simulink library "roblocks"  (R2019a)
settings: Solver=ode45  StartTime=0.0  StopTime=10  RelTol=1e-3  EnableMultiTasking=on
values from neighbouring files (symbols this model uses):
  q = 1    [quadrotor_plot.m]
undefined symbols (not defined in the file or in its folder): a, angdiff, camera, cinertia, cond, delta2tr, eul2tr, fkine, gravload, inertia, jacob0, jacobe, numcols, P, p560, purepursuit, qd, qdd, qz, rne, robot, rpy2tr, tr2delta, tr2eul, tr2rpy, transl, trnorm, trotz, v_max
(part 2 of 2)

== system roblocks/Vision ==
  note: Cameras
  note: Machine vision
  note: Copyright © 2018 Peter Corke
  note: Machine Vision Toolbox
      | for MATLAB®
  Pose estimation : Subsystem  mask{cam=camera, P=P}
      mask prompts: cam "Camera"; P "Points (3xN)"
      mask help: Pose estimation
      mask Help:
      | Estimate pose of an object based on known 3D points with respect to object
      | coordinate frame, a camera model, and observed object point projections.
      | 
      | <b>Parameters::</b>
      | 
      | Camera (Camera)  The camera object, subclass of Camera class
      | Points (3xN)     The 3D world points in object coordinate frame, one per column
      | 
      | <b>Inputs::</b>
      | 
      | Points (2xN)  The 2D image-plane points, one per column, corresponding
      |               to the columns of Points.
      | 
      | <b>Outputs::</b>
      | 
      | T (4x4) the estimated object pose as a homogeneous transformation
      | 
      | <b>Notes::</b>
      | 
      | - A wrapper for the Toolbox method estpose().
  camera : Subsystem  mask{cam=, points=}
      mask prompts: cam "Camera"; points "Points (3xN)"
      mask help: Camera model
      mask Help:
      | A generalized camera model that projects a set of world points to the image
      | plane.
      | 
      | 
      | <b>Parameters::</b>
      | 
      | Camera (Camera)  The camera object, subclass of Camera class
      | Points (3xN)     The 3D world points, one per column
      | 
      | <b>Inputs::</b>
      | 
      | T (4x4) the camera pose as a homogeneous transformation
      | 
      | 
      | <b>Outputs::</b>
      | 
      | p (2xN) projection of world points, one per column, corresponding to columns
      |         of the parameter Points.
      | 
      | <b>Notes::</b>
      | 
      | - Accepts any camera object derived from the abstract Camera superclass.
  camera1 : Subsystem  mask{cam=0}
      mask prompts: cam "Camera"
      mask help: Camera model for moving object
      mask Help:
      | A generalized camera model that projects a set of world points to the image
      | plane.
      | 
      | 
      | <b>Parameters::</b>
      | 
      | Camera (Camera)  The camera object, subclass of Camera class
      | Points (3xN)     The 3D world points, one per column, with respect to the
      |                  object coordinate frame.
      | 
      | <b>Inputs::</b>
      | 
      | T (4x4)    the camera pose as a homogeneous transformation
      | Tobj (4x4) the pose of the object coordinate frame
      | 
      | <b>Outputs::</b>
      | 
      | p (2xN) projection of world points, one per column, corresponding to columns
      |         of the parameter Points.
      | 
      | <b>Notes::</b>
      | 
      | - This block allows for the object to move, as well as the camera.
      | - Accepts any camera object derived from the abstract Camera superclass.
  camera2 : Subsystem  mask{cam=0, points=0}
      mask prompts: cam "Camera"; points "Points (3xN)"
      mask help: Camera model for moving object
      mask Help:
      | A generalized camera model that projects a set of world points to the image
      | plane.
      | 
      | 
      | <b>Parameters::</b>
      | 
      | Camera (Camera)  The camera object, subclass of Camera class
      | Points (3xN)     The 3D world points, one per column, with respect to the
      |                  object coordinate frame.
      | 
      | <b>Inputs::</b>
      | 
      | T (4x4)    the camera pose as a homogeneous transformation
      | Tobj (4x4) the pose of the object coordinate frame
      | 
      | <b>Outputs::</b>
      | 
      | p (2xN) projection of world points, one per column, corresponding to columns
      |         of the parameter Points.
      | 
      | <b>Notes::</b>
      | 
      | - This block allows for the object to move, as well as the camera.
      | - Accepts any camera object derived from the abstract Camera superclass.
  image Jacobian : Subsystem  mask{cam=, z=}
      mask prompts: cam "Camera"; z "Assumed depth (m)"
      mask help: Image Jacobian
      mask Help:
      | Jacobian matrix relating image plane point velocity to camera spatial
      | velocity expressed in the world frame.
      | 
      | <b>Parameters::</b>
      | 
      | Camera (Camera)  The camera object, subclass of Camera class
      | z (1x1)          Point depth, assumed same for all points
      | z (1xN)          Point depth, unique for each point
      | 
      | <b>Inputs::</b>
      | 
      | Points (2xN)     The 2D image-plane points, one per column
      | 
      | 
      | <b>Outputs::</b>
      | 
      | J (2Nx6) the image Jacobian matrix
      | 
      | <b>Notes::</b>
      | 
      | - For multiple points the Jacobian is the "stack" of the 2x6 point feature
      |   Jacobians.
      | - A wrapper for the Toolbox method visjac_p().

== system roblocks/Arm/RNE ==
  q : Inport
  qd : Inport  Port=2
  qdd : Inport  Port=3
  MATLAB Fcn : MATLABFcn  MATLABFcn=rne(robot, u(1:n)', u(n+1:2*n)', u(2*n+1:3*n)')  OutputDimensions=robot.n
  Mux : Mux  Inputs=3
  Q : Outport
  wires:
  Mux/1 -> MATLAB Fcn/1
  q/1 -> Mux/1
  qd/1 -> Mux/2
  qdd/1 -> Mux/3
  MATLAB Fcn/1 -> Q/1

== system roblocks/Arm/Robot ==
  Q : Inport
  Integrator : Integrator
  Integrator1 : Integrator  InitialCondition=q0
  Mux : Mux  Inputs=3
  S-Function : S-Function  FunctionName=slaccel  Parameters=robot  SFunctionDeploymentMode=off  EnableBusSupport=off
  q : Outport
  qd : Outport  Port=2
  qdd : Outport  Port=3
  wires:
  Integrator1/1 -> Mux/1, q/1
  Q/1 -> Mux/3
  Integrator/1 -> Mux/2, Integrator1/1, qd/1  "qd"
  Mux/1 -> S-Function/1
  S-Function/1 -> Integrator/1, qdd/1  "qdd"

== system roblocks/Arm/cinertia ==
  q : Inport
  cinertia : MATLABFcn  MATLABFcn=cinertia(robot,u')  OutputDimensions=[6 6]  Output1D=off
  Alpha : Outport
  wires:
  cinertia/1 -> Alpha/1
  q/1 -> cinertia/1

== system roblocks/Arm/fkine ==
  q : Inport
  MATLAB Fcn : MATLABFcn  MATLABFcn=double(fkine(robot,u))  OutputDimensions=[4 4]  Output1D=off
  T : Outport
  wires:
  MATLAB Fcn/1 -> T/1
  q/1 -> MATLAB Fcn/1

== system roblocks/Arm/gravload ==
  q : Inport
  gravload : MATLABFcn  MATLABFcn=gravload(robot,u')  OutputDimensions=[1 robot.n]  Output1D=off
  g : Outport
  wires:
  gravload/1 -> g/1
  q/1 -> gravload/1

== system roblocks/Arm/ijacob ==
  J : Inport
  inverse jacobian : MATLABFcn  MATLABFcn=inv(u)  Output1D=off
  Ji : Outport
  wires:
  J/1 -> inverse jacobian/1
  inverse jacobian/1 -> Ji/1

== system roblocks/Arm/ikine ==
  T : Inport
  ikine : MATLABFcn  MATLABFcn=robot.ikine(u, q0, M, opt{:})
  q : Outport
  wires:
  T/1 -> ikine/1
  ikine/1 -> q/1

== system roblocks/Arm/ikine6s ==
  T : Inport
  ikine6s : MATLABFcn  MATLABFcn=robot.ikine6s(u,conf)
  q : Outport
  wires:
  T/1 -> ikine6s/1
  ikine6s/1 -> q/1

== system roblocks/Arm/inertia ==
  q : Inport
  inertia : MATLABFcn  MATLABFcn=inertia(robot,u')  OutputDimensions=[robot.n robot.n]  Output1D=off
  J : Outport
  wires:
  inertia/1 -> J/1
  q/1 -> inertia/1

== system roblocks/Arm/jacob0  ==
  q : Inport
  MATLAB Fcn : MATLABFcn  MATLABFcn=jacob0(robot,u)  OutputDimensions=[6 n]  Output1D=off
  J : Outport
  wires:
  q/1 -> MATLAB Fcn/1
  MATLAB Fcn/1 -> J/1

== system roblocks/Arm/jacobn ==
  q : Inport
  MATLAB Fcn : MATLABFcn  MATLABFcn=jacobe(robot,u)  OutputDimensions=[6 n]  Output1D=off
  J : Outport
  wires:
  q/1 -> MATLAB Fcn/1
  MATLAB Fcn/1 -> J/1

== system roblocks/Arm/plot ==
  q : Inport
  S-Function : S-Function  FunctionName=slplotbot  Parameters=robot,fps,holdplot  SFunctionDeploymentMode=off  EnableBusSupport=off
  fps : ZeroOrderHold  SampleTime=1/fps
  wires:
  fps/1 -> S-Function/1
  q/1 -> fps/1

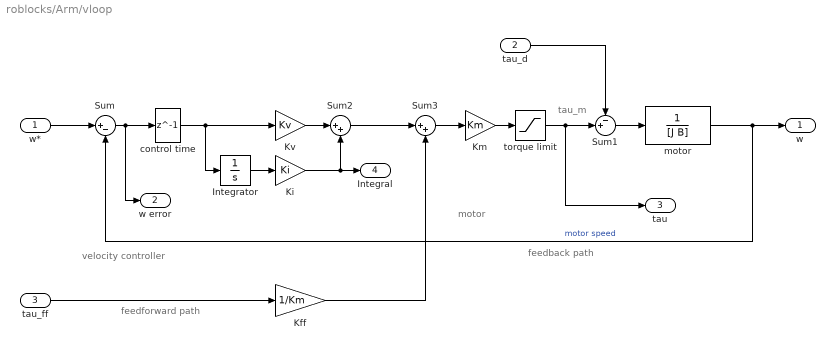
== system roblocks/Arm/vloop ==
  note: feedback path
  note: motor
  note: tau_m
  note: feedforward path
  note: velocity controller
  w* : Inport
  tau_d : Inport  Port=2
  tau_ff : Inport  Port=3
  Integrator : Integrator
  Kff : Gain  Gain=1/Km
  Ki : Gain  Gain=Ki
  Km : Gain  Gain=Km
  Kv : Gain  Gain=Kv
  Sum : Sum  Inputs=|+-
  Sum1 : Sum  Inputs=-+|
  Sum2 : Sum  Inputs=|++
  Sum3 : Sum  Inputs=|++
  control time : Delay  DelayLength=1  SampleTime=T
  motor : TransferFcn  Denominator=[J B]  ContinuousStateAttributes='qd'
  torque limit : Saturate  UpperLimit=tau_max  LowerLimit=-tau_max
  w : Outport
  w error : Outport  Port=2
  tau : Outport  Port=3
  Integral : Outport  Port=4
  wires:
  Sum1/1 -> motor/1
  Sum/1 -> control time/1, w error/1
  motor/1 -> w/1, Sum/2  "motor speed"
  tau_d/1 -> Sum1/1
  torque limit/1 -> Sum1/2, tau/1
  control time/1 -> Kv/1, Integrator/1
  w*/1 -> Sum/1
  Km/1 -> torque limit/1
  Kv/1 -> Sum2/1
  Integrator/1 -> Ki/1
  Ki/1 -> Integral/1, Sum2/2
  Sum2/1 -> Sum3/1
  Sum3/1 -> Km/1
  Kff/1 -> Sum3/2
  tau_ff/1 -> Kff/1

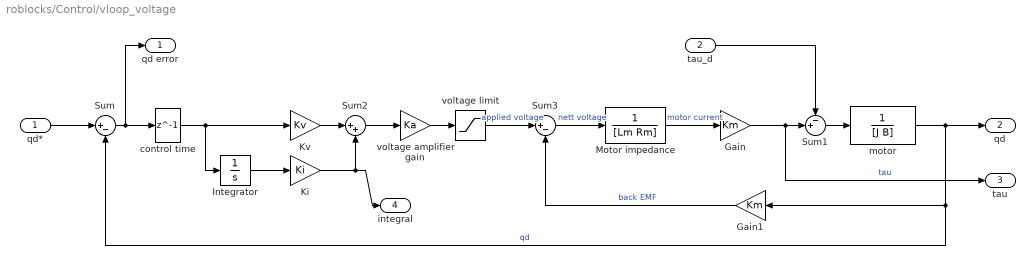
== system roblocks/Control/vloop_voltage ==
  qd* : Inport
  tau_d : Inport  Port=2
  Gain : Gain  Gain=Km
  Gain1 : Gain  Gain=Km
  Integrator : Integrator
  Ki : Gain  Gain=Ki
  Kv : Gain  Gain=Kv
  Motor impedance : TransferFcn  Denominator=[Lm Rm]
  Sum : Sum  Inputs=|+-
  Sum1 : Sum  Inputs=-+|
  Sum2 : Sum  Inputs=|++
  Sum3 : Sum  Inputs=|+-
  control time : Delay  DelayLength=1  SampleTime=T
  motor : TransferFcn  Denominator=[J B]  ContinuousStateAttributes='qd'
  voltage amplifier gain : Gain  Gain=Ka
  voltage limit : Saturate  UpperLimit=v_max  LowerLimit=-v_max
  qd error : Outport
  qd : Outport  Port=2
  tau : Outport  Port=3
  integral : Outport  Port=4
  wires:
  Gain1/1 -> Sum3/2  "back EMF"
  Gain/1 -> tau/1, Sum1/2  "tau"
  Motor impedance/1 -> Gain/1  "motor current"
  Sum3/1 -> Motor impedance/1  "nett voltage"
  voltage limit/1 -> Sum3/1  "applied voltage"
  voltage amplifier gain/1 -> voltage limit/1
  Ki/1 -> integral/1, Sum2/2
  Integrator/1 -> Ki/1
  Kv/1 -> Sum2/1
  Sum2/1 -> voltage amplifier gain/1
  qd*/1 -> Sum/1
  control time/1 -> Integrator/1, Kv/1
  tau_d/1 -> Sum1/1
  motor/1 -> Gain1/1, Sum/2, qd/1  "qd"
  Sum/1 -> qd error/1, control time/1
  Sum1/1 -> motor/1

== system roblocks/Toolbox/Circle ==
  Clock : Clock
  Mux : Mux  Inputs=2
  Product1 : Product  RndMeth=Zero
  Trigonometric Function1 : Trigonometry  Operator=cos
  Trigonometric Function3 : Trigonometry
  freq : Gain  Gain=freq*2*pi
  radius : Constant  Value=radius
  xy : Outport
  wires:
  Trigonometric Function3/1 -> Mux/2
  Trigonometric Function1/1 -> Mux/1
  Mux/1 -> Product1/1
  radius/1 -> Product1/2
  Clock/1 -> freq/1
  Product1/1 -> xy/1
  freq/1 -> Trigonometric Function1/1, Trigonometric Function3/1

== system roblocks/Toolbox/Inverse ==
  T : Inport
  MATLAB Fcn : MATLABFcn  MATLABFcn=inv(u)  OutputDimensions=[4,4]  Output1D=off
  invT : Outport
  wires:
  MATLAB Fcn/1 -> invT/1
  T/1 -> MATLAB Fcn/1

== system roblocks/Toolbox/Post multiply ==
  T1 : Inport
  Constant : Constant  Value=T2
  Product : Product  Multiplication=Matrix(*)  RndMeth=Zero
  T : Outport
  wires:
  T1/1 -> Product/1
  Constant/1 -> Product/2
  Product/1 -> T/1

== system roblocks/Toolbox/Pre multiply ==
  T2 : Inport
  Constant : Constant  Value=T  VectorParams1D=off
  Product : Product  Multiplication=Matrix(*)  RndMeth=Zero
  T : Outport
  wires:
  T2/1 -> Product/2
  Product/1 -> T/1
  Constant/1 -> Product/1

== system roblocks/Toolbox/SE2 to SE3 ==
  SE2 : Inport
  SE2->SE3 : MATLABFcn  MATLABFcn=transl(u(1), u(2), 0)*trotz(u(3))  Output1D=off
  T : Outport
  wires:
  SE2->SE3/1 -> T/1
  SE2/1 -> SE2->SE3/1

== system roblocks/Toolbox/T2eul ==
  T : Inport
  Demux : Demux  Outputs=3
  MATLAB Fcn : MATLABFcn  MATLABFcn=tr2eul(u, args{:})  OutputDimensions=3
  a : Outport
  b : Outport  Port=2
  c : Outport  Port=3
  wires:
  T/1 -> MATLAB Fcn/1
  MATLAB Fcn/1 -> Demux/1
  Demux/1 -> a/1
  Demux/2 -> b/1
  Demux/3 -> c/1

== system roblocks/Toolbox/T2rpy ==
  T : Inport
  Demux : Demux  Outputs=3
  MATLAB Fcn : MATLABFcn  MATLABFcn=tr2rpy(u, args{:})  OutputDimensions=3
  roll : Outport
  pitch : Outport  Port=2
  yaw : Outport  Port=3
  wires:
  T/1 -> MATLAB Fcn/1
  MATLAB Fcn/1 -> Demux/1
  Demux/1 -> roll/1
  Demux/2 -> pitch/1
  Demux/3 -> yaw/1

== system roblocks/Toolbox/T2xyz ==
  T : Inport
  Demux : Demux  Outputs=3
  MATLAB Fcn : MATLABFcn  MATLABFcn=transl(u)  OutputDimensions=3
  x : Outport
  y : Outport  Port=2
  z : Outport  Port=3
  wires:
  Demux/3 -> z/1
  Demux/2 -> y/1
  Demux/1 -> x/1
  MATLAB Fcn/1 -> Demux/1
  T/1 -> MATLAB Fcn/1

== system roblocks/Toolbox/angdiff ==
  + : Inport
  - : Inport  Port=2
  MATLAB Fcn : MATLABFcn  MATLABFcn=angdiff(u(1), u(2))
  Mux : Mux  Inputs=2
  d : Outport
  wires:
  -/1 -> Mux/2
  MATLAB Fcn/1 -> d/1
  Mux/1 -> MATLAB Fcn/1
  +/1 -> Mux/1

== system roblocks/Toolbox/angdiff1 ==
  + : Inport
  MATLAB Fcn : MATLABFcn  MATLABFcn=angdiff(u)
  d : Outport
  wires:
  MATLAB Fcn/1 -> d/1
  +/1 -> MATLAB Fcn/1

== system roblocks/Toolbox/eul2T ==
  a : Inport
  b : Inport  Port=2
  c : Inport  Port=3
  MATLAB Fcn : MATLABFcn  MATLABFcn=eul2tr(u', args{:})  OutputDimensions=[4 4]  Output1D=off
  Mux : Mux  Inputs=3
  T : Outport
  wires:
  b/1 -> Mux/2
  a/1 -> Mux/1
  Mux/1 -> MATLAB Fcn/1
  MATLAB Fcn/1 -> T/1
  c/1 -> Mux/3

== system roblocks/Toolbox/invJac ==
  J : Inport
  e : Inport  Port=2
  MATLAB Fcn2 : MATLABFcn  MATLABFcn=cond(u)  Output1D=off
  Product1 : Product  Multiplication=Matrix(*)  SaturateOnIntegerOverflow=on  RndMeth=Zero  InputSameDT=on  OutDataTypeStr=Inherit: Same as first input
  inv : MATLABFcn  MATLABFcn=pinv(u)  Output1D=off
  vdot : Outport
  cond : Outport  Port=2
  wires:
  Product1/1 -> vdot/1
  MATLAB Fcn2/1 -> cond/1
  e/1 -> Product1/2
  inv/1 -> Product1/1
  J/1 -> inv/1, MATLAB Fcn2/1

== system roblocks/Toolbox/jtraj ==
  Clock : Clock
  MATLAB Fcn : MATLABFcn  MATLABFcn=interp1(t,q,min(u,tmax))  OutputDimensions=n  SampleTime=ts
  MATLAB Fcn1 : MATLABFcn  MATLABFcn=interp1(t,qd,min(u,tmax))  OutputDimensions=n  SampleTime=ts
  MATLAB Fcn2 : MATLABFcn  MATLABFcn=interp1(t,qdd,min(u,tmax))  OutputDimensions=n  SampleTime=ts
  q : Outport
  qd : Outport  Port=2
  qdd : Outport  Port=3
  wires:
  MATLAB Fcn2/1 -> qdd/1
  Clock/1 -> MATLAB Fcn2/1, MATLAB Fcn1/1, MATLAB Fcn/1
  MATLAB Fcn1/1 -> qd/1
  MATLAB Fcn/1 -> q/1

== system roblocks/Toolbox/lspb ==
  Clock : Clock
  MATLAB Fcn : MATLABFcn  MATLABFcn=interp1(t,q,u)  OutputDimensions=n
  MATLAB Fcn1 : MATLABFcn  MATLABFcn=interp1(t,qd,u)  OutputDimensions=n
  MATLAB Fcn2 : MATLABFcn  MATLABFcn=interp1(t,qdd,u)  OutputDimensions=n
  q : Outport
  qd : Outport  Port=2
  qdd : Outport  Port=3
  wires:
  MATLAB Fcn/1 -> q/1
  MATLAB Fcn1/1 -> qd/1
  Clock/1 -> MATLAB Fcn/1, MATLAB Fcn1/1, MATLAB Fcn2/1
  MATLAB Fcn2/1 -> qdd/1

== system roblocks/Toolbox/mstraj ==
  Clock : Clock
  Interpreted MATLAB Function : MATLABFcn  MATLABFcn=interp1( linspace(0, total_time, size(robot_traj,1)), robot_traj, u)
  xy : Outport
  wires:
  Clock/1 -> Interpreted MATLAB Function/1
  Interpreted MATLAB Function/1 -> xy/1

== system roblocks/Toolbox/norm ==
  v : Inport
  norm : MATLABFcn  MATLABFcn=norm(u)
  n : Outport
  wires:
  norm/1 -> n/1
  v/1 -> norm/1

== system roblocks/Toolbox/pinvJac ==
  J : Inport
  e : Inport  Port=2
  MATLAB Fcn2 : MATLABFcn  MATLABFcn=cond(u)  Output1D=off
  Product1 : Product  Multiplication=Matrix(*)  SaturateOnIntegerOverflow=on  RndMeth=Zero  InputSameDT=on  OutDataTypeStr=Inherit: Same as first input
  pinv : MATLABFcn  MATLABFcn=pinv(u)  Output1D=off
  vdot : Outport
  cond : Outport  Port=2
  wires:
  Product1/1 -> vdot/1
  MATLAB Fcn2/1 -> cond/1
  e/1 -> Product1/2
  pinv/1 -> Product1/1
  J/1 -> pinv/1, MATLAB Fcn2/1

== system roblocks/Toolbox/pose integral ==
  v : Inport
  MATLAB Fcn3 : MATLABFcn  MATLABFcn=delta2tr(u*dt)  Output1D=off
  Product : Product  Multiplication=Matrix(*)  RndMeth=Zero
  Unit Delay : UnitDelay  InitialCondition=T0  SampleTime=dt  HasFrameUpgradeWarning=on
  trnorm : MATLABFcn  MATLABFcn=trnorm(u)  Output1D=off
  T : Outport
  wires:
  v/1 -> MATLAB Fcn3/1
  trnorm/1 -> Unit Delay/1
  MATLAB Fcn3/1 -> Product/1
  Unit Delay/1 -> T/1, Product/2
  Product/1 -> trnorm/1

== system roblocks/Toolbox/pure pursuit ==
  CP : Inport
  Interpreted MATLAB Function : MATLABFcn  MATLABFcn=purepursuit(u, R, robot_traj)
  PP : Outport
  wires:
  CP/1 -> Interpreted MATLAB Function/1
  Interpreted MATLAB Function/1 -> PP/1

== system roblocks/Toolbox/rpy2T ==
  roll : Inport
  pitch : Inport  Port=2
  yaw : Inport  Port=3
  MATLAB Fcn : MATLABFcn  MATLABFcn=rpy2tr(u', args{:})  OutputDimensions=[4 4]  Output1D=off
  Mux : Mux  Inputs=3
  T : Outport
  wires:
  pitch/1 -> Mux/2
  roll/1 -> Mux/1
  Mux/1 -> MATLAB Fcn/1
  MATLAB Fcn/1 -> T/1
  yaw/1 -> Mux/3

== system roblocks/Toolbox/tr2delta ==
  T1 : Inport
  T2 : Inport  Port=2
  MATLAB Fcn : MATLABFcn  MATLABFcn=tr2delta(reshape(u(1:16),4,4), reshape(u(17:32),4,4))  OutputDimensions=6
  Mux : Mux  Inputs=2
  Reshape : Reshape
  Reshape1 : Reshape
  delta : Outport
  wires:
  Reshape1/1 -> Mux/2
  Reshape/1 -> Mux/1
  Mux/1 -> MATLAB Fcn/1
  T2/1 -> Reshape1/1
  T1/1 -> Reshape/1
  MATLAB Fcn/1 -> delta/1

== system roblocks/Toolbox/tr2diff ==
  T1 : Inport
  T2 : Inport  Port=2
  MATLAB Fcn : MATLABFcn  MATLABFcn=tr2delta(reshape(u(1:16),4,4), reshape(u(17:32),4,4))  OutputDimensions=6
  Mux : Mux  Inputs=2
  Reshape : Reshape
  Reshape1 : Reshape
  dx : Outport
  wires:
  Reshape1/1 -> Mux/2
  Reshape/1 -> Mux/1
  Mux/1 -> MATLAB Fcn/1
  T2/1 -> Reshape1/1
  T1/1 -> Reshape/1
  MATLAB Fcn/1 -> dx/1

== system roblocks/Toolbox/trprint ==
  T : Inport
  S-Function : S-Function  FunctionName=sltrprint  Parameters=options  SFunctionDeploymentMode=off  EnableBusSupport=off
  wires:
  T/1 -> S-Function/1

== system roblocks/Toolbox/xyt to SE3 ==
  x : Inport
  y : Inport  Port=2
  theta : Inport  Port=3
  Mux : Mux  Inputs=3
  SE2->SE3 : MATLABFcn  MATLABFcn=transl(u(1), u(2), 0)*trotz(u(3))  Output1D=off
  T : Outport
  wires:
  Mux/1 -> SE2->SE3/1
  y/1 -> Mux/2
  x/1 -> Mux/1
  theta/1 -> Mux/3
  SE2->SE3/1 -> T/1

== system roblocks/Toolbox/xyz2T ==
  x : Inport
  y : Inport  Port=2
  z : Inport  Port=3
  MATLAB Fcn : MATLABFcn  MATLABFcn=transl(u)  OutputDimensions=[4 4]  Output1D=off
  Mux : Mux  Inputs=3
  T : Outport
  wires:
  z/1 -> Mux/3
  MATLAB Fcn/1 -> T/1
  Mux/1 -> MATLAB Fcn/1
  x/1 -> Mux/1
  y/1 -> Mux/2

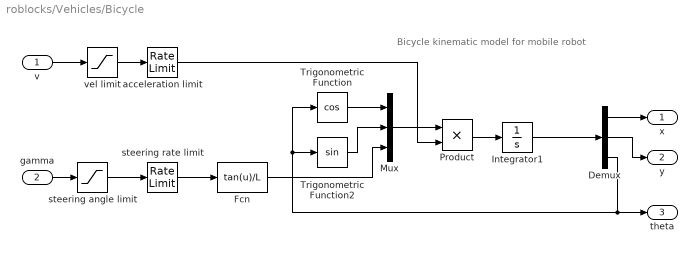
== system roblocks/Vehicles/Bicycle ==
  note: Bicycle kinematic model for mobile robot
  v : Inport
  gamma : Inport  Port=2
  Demux : Demux  Outputs=3
  Fcn : Fcn  Expr=tan(u)/L
  Integrator1 : Integrator  InitialCondition=x0
  Mux : Mux  Inputs=3
  Product : Product  RndMeth=Zero
  Trigonometric Function : Trigonometry  Operator=cos
  Trigonometric Function2 : Trigonometry
  acceleration limit : RateLimiter  RisingSlewLimit=accel  FallingSlewLimit=-accel  SampleTimeMode=inherited
  steering angle limit : Saturate  UpperLimit=alim  LowerLimit=-alim
  steering rate limit : RateLimiter  RisingSlewLimit=steer_rate  FallingSlewLimit=-steer_rate  SampleTimeMode=inherited
  vel limit : Saturate  UpperLimit=vlim  LowerLimit=-vlim
  x : Outport
  y : Outport  Port=2
  theta : Outport  Port=3
  wires:
  steering angle limit/1 -> steering rate limit/1
  Trigonometric Function2/1 -> Mux/2
  vel limit/1 -> acceleration limit/1
  Mux/1 -> Product/1
  v/1 -> vel limit/1
  gamma/1 -> steering angle limit/1
  Demux/2 -> y/1
  Demux/1 -> x/1
  Demux/3 -> theta/1, Trigonometric Function2/1, Trigonometric Function/1
  acceleration limit/1 -> Product/2
  Trigonometric Function/1 -> Mux/1
  Fcn/1 -> Mux/3
  Integrator1/1 -> Demux/1
  Product/1 -> Integrator1/1
  steering rate limit/1 -> Fcn/1

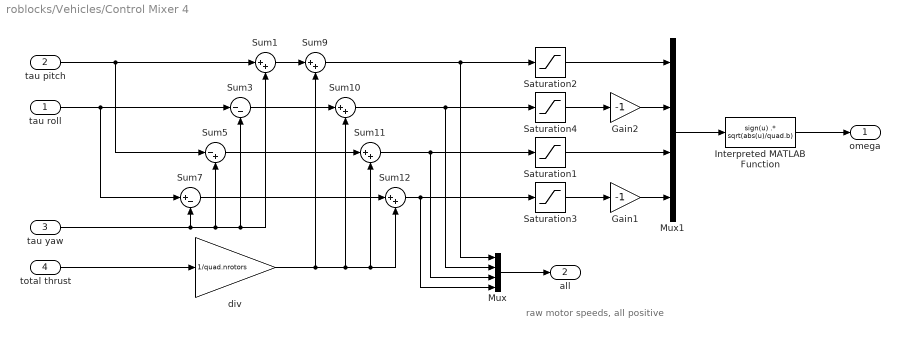
== system roblocks/Vehicles/Control Mixer 4 ==
  note: raw motor speeds, all positive
  tau roll : Inport
  tau pitch : Inport  Port=2
  tau yaw : Inport  Port=3
  total thrust : Inport  Port=4
  Gain1 : Gain  Gain=-1
  Gain2 : Gain  Gain=-1
  Interpreted MATLAB Function : MATLABFcn  MATLABFcn=sign(u) .* sqrt(abs(u)/quad.b)
  Mux : Mux
  Mux1 : Mux
  Saturation{1..4} (4 alike) : Saturate  UpperLimit=maxrot  LowerLimit=minrot
  Sum{1,9..12} (5 alike) : Sum  Inputs=|++  SaturateOnIntegerOverflow=on  InputSameDT=on  OutDataTypeStr=Inherit: Same as first input
  Sum3 : Sum  Inputs=|--  SaturateOnIntegerOverflow=on  InputSameDT=on  OutDataTypeStr=Inherit: Same as first input
  Sum5 : Sum  Inputs=|-+  SaturateOnIntegerOverflow=on  InputSameDT=on  OutDataTypeStr=Inherit: Same as first input
  Sum7 : Sum  Inputs=|+-  SaturateOnIntegerOverflow=on  InputSameDT=on  OutDataTypeStr=Inherit: Same as first input
  div : Gain  Gain=1/quad.nrotors
  omega : Outport
  all : Outport  Port=2
  wires:
  Gain1/1 -> Mux1/4
  Mux/1 -> all/1
  tau roll/1 -> Sum7/1, Sum3/1
  total thrust/1 -> div/1
  Sum12/1 -> Saturation3/1, Mux/4
  Sum11/1 -> Saturation1/1, Mux/3
  Sum10/1 -> Saturation4/1, Mux/2
  Sum9/1 -> Mux/1, Saturation2/1
  Sum7/1 -> Sum12/1
  Sum5/1 -> Sum11/1
  Sum3/1 -> Sum10/1
  Sum1/1 -> Sum9/1
  tau pitch/1 -> Sum5/1, Sum1/1
  Saturation3/1 -> Gain1/1
  Saturation1/1 -> Mux1/3
  Saturation4/1 -> Gain2/1
  Saturation2/1 -> Mux1/1
  tau yaw/1 -> Sum1/2, Sum3/2, Sum5/2, Sum7/2
  Gain2/1 -> Mux1/2
  Mux1/1 -> Interpreted MATLAB Function/1
  Interpreted MATLAB Function/1 -> omega/1
  div/1 -> Sum9/2, Sum10/2, Sum12/2, Sum11/2

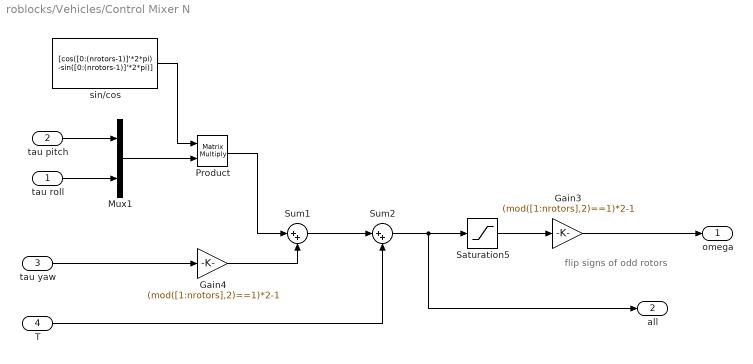
== system roblocks/Vehicles/Control Mixer N ==
  note: flip signs of odd rotors
  tau roll : Inport
  tau pitch : Inport  Port=2
  tau yaw : Inport  Port=3
  T : Inport  Port=4
  Gain3 : Gain  Gain=(mod([1:nrotors],2)==1)*2-1
  Gain4 : Gain  Gain=(mod([1:nrotors],2)==1)*2-1
  Mux1 : Mux  Inputs=2
  Product : Product  Multiplication=Matrix(*)
  Saturation5 : Saturate  UpperLimit=wmax  LowerLimit=wmin
  Sum1 : Sum  Inputs=|++  SaturateOnIntegerOverflow=on  InputSameDT=on  OutDataTypeStr=Inherit: Same as first input
  Sum2 : Sum  Inputs=|++  SaturateOnIntegerOverflow=on  InputSameDT=on  OutDataTypeStr=Inherit: Same as first input
  sin/cos : Constant  Value="[cos([0:(nrotors-1)]'*2*pi)  -sin([0:(nrotors-1)]'*2*pi)]"  VectorParams1D=off  SampleTime=0
  omega : Outport
  all : Outport  Port=2
  wires:
  tau roll/1 -> Mux1/2
  Sum2/1 -> all/1, Saturation5/1
  Saturation5/1 -> Gain3/1
  T/1 -> Sum2/2
  Sum1/1 -> Sum2/1
  tau yaw/1 -> Gain4/1
  Gain4/1 -> Sum1/2
  Gain3/1 -> omega/1
  tau pitch/1 -> Mux1/1
  Mux1/1 -> Product/2
  sin/cos/1 -> Product/1
  Product/1 -> Sum1/1

== system roblocks/Vehicles/N-rotor ==
  omega : Inport
  Bus Creator : BusCreator  Inputs='X','Y','Z','yaw','pitch','roll','dx','dy','dz','dyaw','dpitch','droll'
  Demux : Demux  Outputs=12
  Dynamics : S-Function  FunctionName=nrotor_dynamics  Parameters=quad, x0, ground  SFunctionDeploymentMode=off  EnableBusSupport=off
  X : Outport
  wires:
  Demux/12 -> Bus Creator/12  "droll"
  Demux/11 -> Bus Creator/11  "dpitch"
  Demux/10 -> Bus Creator/10  "dyaw"
  Dynamics/1 -> Demux/1
  Bus Creator/1 -> X/1
  Demux/8 -> Bus Creator/8  "dy"
  Demux/6 -> Bus Creator/6  "roll"
  Demux/2 -> Bus Creator/2  "Y"
  Demux/9 -> Bus Creator/9  "dz"
  Demux/7 -> Bus Creator/7  "dx"
  omega/1 -> Dynamics/1
  Demux/5 -> Bus Creator/5  "pitch"
  Demux/4 -> Bus Creator/4  "yaw"
  Demux/3 -> Bus Creator/3  "Z"
  Demux/1 -> Bus Creator/1  "X"

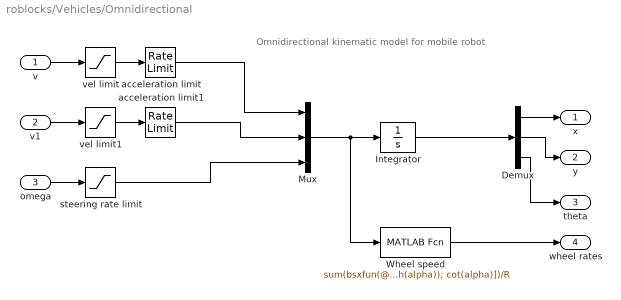
== system roblocks/Vehicles/Omnidirectional ==
  note: Omnidirectional kinematic model for mobile robot
  v : Inport
  v1 : Inport  Port=2
  omega : Inport  Port=3
  Demux : Demux  Outputs=3
  Integrator : Integrator  InitialCondition=x0
  Mux : Mux  Inputs=3
  Wheel speed : MATLABFcn  MATLABFcn=sum(bsxfun(@minus, u(1:2), skew(u(3))*P) .* [ones(1,length(alpha)); cot(alpha)])/R
  acceleration limit : RateLimiter  RisingSlewLimit=accel  FallingSlewLimit=-accel  SampleTimeMode=inherited
  acceleration limit1 : RateLimiter  RisingSlewLimit=accel  FallingSlewLimit=-accel  SampleTimeMode=inherited
  steering rate limit : Saturate  UpperLimit=alim  LowerLimit=-alim
  vel limit : Saturate  UpperLimit=vlim  LowerLimit=-vlim
  vel limit1 : Saturate  UpperLimit=vlim  LowerLimit=-vlim
  x : Outport
  y : Outport  Port=2
  theta : Outport  Port=3
  wheel rates : Outport  Port=4
  wires:
  acceleration limit/1 -> Mux/1
  Demux/3 -> theta/1
  Demux/1 -> x/1
  Demux/2 -> y/1
  omega/1 -> steering rate limit/1
  v/1 -> vel limit/1
  vel limit/1 -> acceleration limit/1
  Mux/1 -> Wheel speed/1, Integrator/1
  Integrator/1 -> Demux/1
  Wheel speed/1 -> wheel rates/1
  v1/1 -> vel limit1/1
  vel limit1/1 -> acceleration limit1/1
  acceleration limit1/1 -> Mux/2
  steering rate limit/1 -> Mux/3

== system roblocks/Vehicles/Quadrotor ==
  omega : Inport
  Bus Creator : BusCreator  Inputs='X','Y','Z','yaw','pitch','roll','dx','dy','dz','dyaw','dpitch','droll'
  Demux : Demux  Outputs=12
  Dynamics : S-Function  FunctionName=quadrotor_dynamics  Parameters=quad, x0, groundflag  SFunctionDeploymentMode=off  EnableBusSupport=off
  X : Outport
  wires:
  Demux/12 -> Bus Creator/12  "droll"
  Demux/11 -> Bus Creator/11  "dpitch"
  Demux/10 -> Bus Creator/10  "dyaw"
  Dynamics/1 -> Demux/1
  Bus Creator/1 -> X/1
  Demux/8 -> Bus Creator/8  "dy"
  Demux/6 -> Bus Creator/6  "roll"
  Demux/2 -> Bus Creator/2  "Y"
  Demux/9 -> Bus Creator/9  "dz"
  Demux/7 -> Bus Creator/7  "dx"
  omega/1 -> Dynamics/1
  Demux/5 -> Bus Creator/5  "pitch"
  Demux/4 -> Bus Creator/4  "yaw"
  Demux/3 -> Bus Creator/3  "Z"
  Demux/1 -> Bus Creator/1  "X"

== system roblocks/Vehicles/Quadrotor plot ==
  X : Inport
  Bus Selector1 : BusSelector  OutputSignals=X,Y,Z,yaw,pitch,roll  OutputAsBus=on
  Plotter : S-Function  FunctionName=quadrotor_plot  Parameters=[xydim, zdim], 1, 1,quad  SFunctionDeploymentMode=off  EnableBusSupport=off
  wires:
  Bus Selector1/1 -> Plotter/1
  X/1 -> Bus Selector1/1

== system roblocks/Vehicles/Tracking controller ==
  xdot : Inport
  ydot : Inport  Port=2
  theta : Inport  Port=3
  Demux : Demux  Outputs=2
  Interpreted MATLAB Function : MATLABFcn  MATLABFcn=[cos(u(3)) sin(u(3)); -1/a*sin(u(3)) 1/a*cos(u(3))] * u(1:2)
  Mux : Mux  Inputs=3
  v : Outport
  omega : Outport  Port=2
  wires:
  Mux/1 -> Interpreted MATLAB Function/1
  Interpreted MATLAB Function/1 -> Demux/1
  theta/1 -> Mux/3
  Demux/2 -> omega/1
  Demux/1 -> v/1
  ydot/1 -> Mux/2
  xdot/1 -> Mux/1

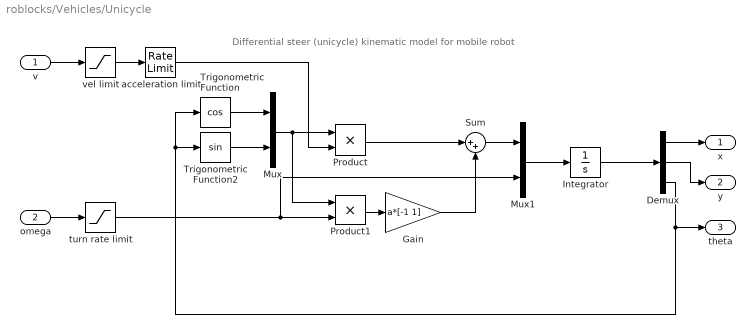
== system roblocks/Vehicles/Unicycle ==
  note: Differential steer (unicycle) kinematic model for mobile robot
  v : Inport
  omega : Inport  Port=2
  Demux : Demux  Outputs=3
  Gain : Gain  Gain=a*[-1 1]
  Integrator : Integrator  InitialCondition=x0
  Mux : Mux  Inputs=2
  Mux1 : Mux  Inputs=2
  Product : Product  RndMeth=Zero
  Product1 : Product  RndMeth=Zero
  Sum : Sum  Inputs=|++
  Trigonometric Function : Trigonometry  Operator=cos
  Trigonometric Function2 : Trigonometry
  acceleration limit : RateLimiter  RisingSlewLimit=alim  FallingSlewLimit=-alim  SampleTimeMode=inherited
  turn rate limit : Saturate  UpperLimit=wlim  LowerLimit=-wlim
  vel limit : Saturate  UpperLimit=vlim  LowerLimit=-vlim
  x : Outport
  y : Outport  Port=2
  theta : Outport  Port=3
  wires:
  Trigonometric Function/1 -> Mux/1
  acceleration limit/1 -> Product/2
  Integrator/1 -> Demux/1
  Demux/3 -> Trigonometric Function/1, Trigonometric Function2/1, theta/1
  Demux/1 -> x/1
  Demux/2 -> y/1
  omega/1 -> turn rate limit/1
  v/1 -> vel limit/1
  Mux/1 -> Product1/1, Product/1
  vel limit/1 -> acceleration limit/1
  Trigonometric Function2/1 -> Mux/2
  turn rate limit/1 -> Mux1/2, Product1/2
  Mux1/1 -> Integrator/1
  Product/1 -> Sum/1
  Sum/1 -> Mux1/1
  Product1/1 -> Gain/1
  Gain/1 -> Sum/2

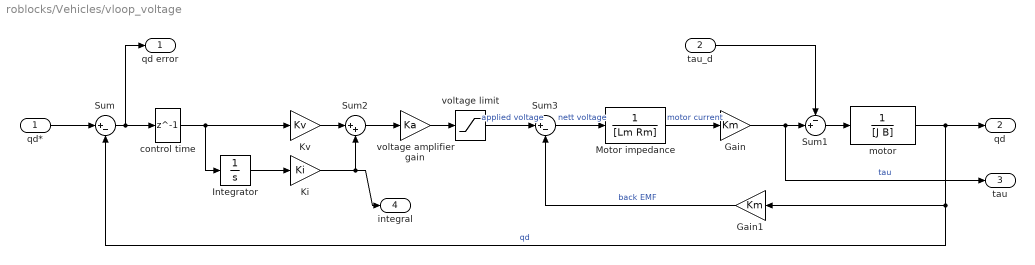
== system roblocks/Vehicles/vloop_voltage ==
  qd* : Inport
  tau_d : Inport  Port=2
  Gain : Gain  Gain=Km
  Gain1 : Gain  Gain=Km
  Integrator : Integrator
  Ki : Gain  Gain=Ki
  Kv : Gain  Gain=Kv
  Motor impedance : TransferFcn  Denominator=[Lm Rm]
  Sum : Sum  Inputs=|+-
  Sum1 : Sum  Inputs=-+|
  Sum2 : Sum  Inputs=|++
  Sum3 : Sum  Inputs=|+-
  control time : Delay  DelayLength=1  SampleTime=T
  motor : TransferFcn  Denominator=[J B]  ContinuousStateAttributes='qd'
  voltage amplifier gain : Gain  Gain=Ka
  voltage limit : Saturate  UpperLimit=v_max  LowerLimit=-v_max
  qd error : Outport
  qd : Outport  Port=2
  tau : Outport  Port=3
  integral : Outport  Port=4
  wires:
  Sum1/1 -> motor/1
  Sum/1 -> control time/1, qd error/1
  motor/1 -> qd/1, Sum/2, Gain1/1  "qd"
  tau_d/1 -> Sum1/1
  control time/1 -> Kv/1, Integrator/1
  qd*/1 -> Sum/1
  Sum2/1 -> voltage amplifier gain/1
  Kv/1 -> Sum2/1
  Integrator/1 -> Ki/1
  Ki/1 -> Sum2/2, integral/1
  voltage amplifier gain/1 -> voltage limit/1
  voltage limit/1 -> Sum3/1  "applied voltage"
  Sum3/1 -> Motor impedance/1  "nett voltage"
  Motor impedance/1 -> Gain/1  "motor current"
  Gain/1 -> Sum1/2, tau/1  "tau"
  Gain1/1 -> Sum3/2  "back EMF"

== system roblocks/Vision/Pose estimation ==
  p : Inport
  MATLAB Fcn : MATLABFcn  MATLABFcn=cam.estpose(P, u).T  OutputDimensions=[4,4]  Output1D=off
  T : Outport
  wires:
  MATLAB Fcn/1 -> T/1
  p/1 -> MATLAB Fcn/1

== system roblocks/Vision/camera ==
  T : Inport
  MATLAB Fcn : MATLABFcn  MATLABFcn=cam.plot(points, 'Tcam', u)  OutputSignalType=real  Output1D=off
  p : Outport
  wires:
  T/1 -> MATLAB Fcn/1
  MATLAB Fcn/1 -> p/1

== system roblocks/Vision/camera1 ==
  T : Inport
  P : Inport  Port=2
  MATLAB Fcn : MATLABFcn  MATLABFcn=slcamera(cam, u)  OutputSignalType=real  Output1D=off
  Mux : Mux  Inputs=2
  Reshape1 : Reshape  OutputDimensionality=Column vector (2-D)  OutputDimensions=6
  Reshape2 : Reshape  OutputDimensionality=Column vector (2-D)  OutputDimensions=6
  p : Outport
  wires:
  MATLAB Fcn/1 -> p/1
  Mux/1 -> MATLAB Fcn/1
  T/1 -> Reshape2/1
  P/1 -> Reshape1/1
  Reshape2/1 -> Mux/1
  Reshape1/1 -> Mux/2

== system roblocks/Vision/camera2 ==
  T : Inport
  Tobj : Inport  Port=2
  MATLAB Fcn : MATLABFcn  MATLABFcn=cam.plot(points, 'Tcam', u(:,:,1), 'Tobj', u(:,:,2), 'drawnow')  OutputDimensions=[2,numcols(points)]  OutputSignalType=real  Output1D=off
  Matrix Concatenate : Concatenate  Mode=Multidimensional array  ConcatenateDimension=3
  p : Outport
  wires:
  T/1 -> Matrix Concatenate/1
  Tobj/1 -> Matrix Concatenate/2
  Matrix Concatenate/1 -> MATLAB Fcn/1
  MATLAB Fcn/1 -> p/1

== system roblocks/Vision/image Jacobian ==
  p : Inport
  MATLAB Fcn : MATLABFcn  MATLABFcn=cam.visjac_p(u, z)  Output1D=off
  J : Outport
  wires:
  p/1 -> MATLAB Fcn/1
  MATLAB Fcn/1 -> J/1
